simulink model "smart_sensor_Simulation"  (Simulink 6.4)
settings: Solver=FixedStepDiscrete  StartTime=0.0  StopTime=10.0  FixedStep=0.001  RelTol=1e-3
libraries: dsPICdrivers x1, simulink x1
settings Model: Creator=Zion  LastModifiedBy=Lubin
settings OptimizationCC: ExpressionDepthLimit=2147483647  OptimizeModelRefInitCode=on  LifeSpan=1  SimCompilerOptimization=Off
settings DebuggingCC: SignalResolutionControl=UseLocalSettings  MultiTaskDSMMsg=error  MultiTaskCondExecSysMsg=error  StateNameClashWarn=warning
settings HardwareCC: ProdBitPerInt=16  ProdEndianess=LittleEndian  ProdWordSize=16  ProdHWDeviceType=16-bit Generic  TargetHWDeviceType=32-bit Generic
settings RTWCC: SystemTargetFile=dspic.tlc  TemplateMakefile=dspic_pic30_gcc.tmf  PostCodeGenCommand=dsPIC_Compile()  Description=Embedded Target for Microchip dsPIC (real-time)  ProcessScript=dspic_make_rtw_hook  RTWCompilerOptimization=Off
settings CodeAppCC: IgnoreCustomStorageClasses=off
settings STFCustomTargetCC: TargetFcnLib=ansi_tfl_tmw.mat  GenFloatMathFcnCalls=ANSI_C  ModelReferenceCompliant=off  IncludeMdlTerminateFcn=off  CombineOutputUpdateFcns=on  SuppressErrorStatus=on  ERTCustomFileBanners=on  SupportContinuousTime=off  SupportNonInlinedSFcns=off  SystemTargetFile=dspic.tlc
settings ERTTargetCC: TargetFcnLib=ansi_tfl_tmw.mat  GenFloatMathFcnCalls=ANSI_C  ModelReferenceCompliant=off  CompOptLevelCompliant=off  IncludeMdlTerminateFcn=off  SuppressErrorStatus=on  ModelStepFunctionPrototypeControlCompliant=off  InlinedParameterPlacement=NonHierarchical  ERTSrcFileBannerTemplate=dsPIC_code_template.cgt  ERTHdrFileBannerTemplate=dsPIC_code_template.cgt  ERTDataSrcFileTemplate=dsPIC_code_template.cgt  ERTDataHdrFileTemplate=dsPIC_code_template.cgt  ERTCustomFileTemplate=dsPIC_main.tlc
settings CustomProperty: DataType=string  Value=C:\PROGRA~1\MATLAB\R2007b\bin\win32\gmake

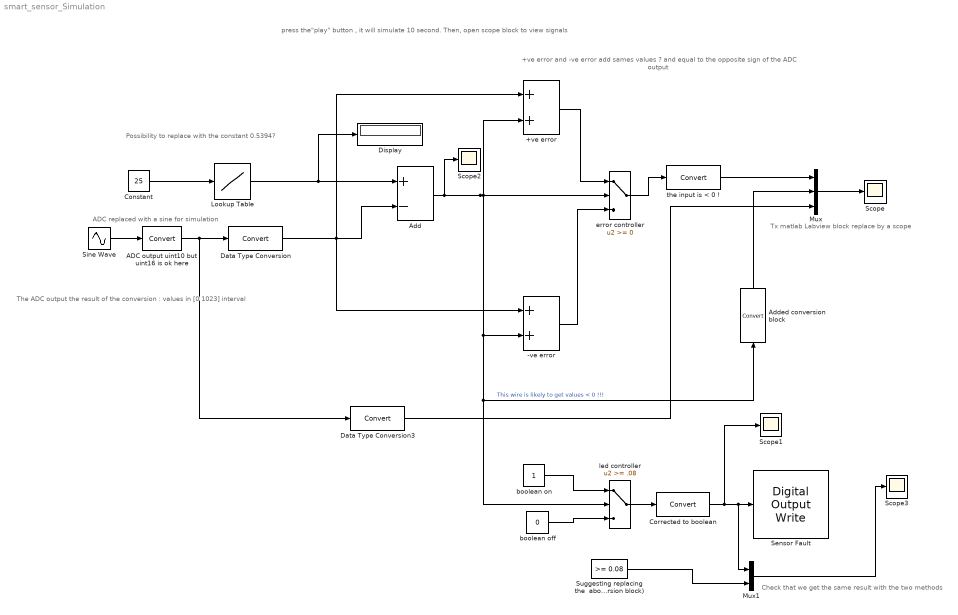
== system smart_sensor_Simulation ==
  note: Possibility to replace with the constant 0.5394?
  note: The ADC output the
      | result of the conversion :
      | values in [0 1023] interval
  note: +ve error and -ve error add sames values ?
      | and equal to the opposite sign of the ADC output
  note: press the"play" button , it will simulate 10 second. Then, open scope block to view signals
  note: ADC replaced with a sine for simulation
  note: Tx matlab Labview block replace by a scope
  note: Check that we get the same result with the two methods
  +ve error : Sum  OutDataTypeMode=double  OutDataType=sfix(16)  OutScaling=2^-10
  -ve error : Sum  OutDataTypeMode=double  OutDataType=sfix(16)  OutScaling=2^-10
  ADC output uint10 but uint16 is ok here : DataTypeConversion  OutDataTypeMode=uint16  OutDataType=sfix(16)  OutScaling=2^0
  Add : Sum  Inputs=+-  OutDataType=sfix(16)  OutScaling=2^-10
  Added conversion block : DataTypeConversion  Orientation=up  OutDataTypeMode=uint16  OutDataType=sfix(16)  OutScaling=2^0
  Constant : Constant  Value=25  OutDataTypeMode=double  OutDataType=sfix(16)  OutScaling=2^0
  Corrected to boolean : DataTypeConversion  OutDataTypeMode=boolean  OutDataType=sfix(16)  OutScaling=2^0
  Data Type Conversion : DataTypeConversion  OutDataTypeMode=double  OutDataType=sfix(16)  OutScaling=2^0
  Data Type Conversion3 : DataTypeConversion  OutDataTypeMode=uint16  OutDataType=sfix(16)  OutScaling=2^0
  Display : Display
  Lookup Table : Lookup  InputValues=[-55 23 150]  OutputValues=[-1.1 .5 3]  LookUpMeth=Interpolation-Use End Values  OutDataTypeMode=double  OutDataType=sfix(16)  OutScaling=2^0
  Mux : Mux  Inputs=3
  Mux1 : Mux  Inputs=2
  Scope{,1..3} (4 alike) : Scope
      Scope2 settings: SaveName=ScopeData2
      Scope3 settings: SaveName=ScopeData3
  Sensor Fault : dsPICdrivers/Digital I//O/Digital Output Write  Tag=dsPIC_Digital_Output  Priority=5  PORT=E  Pin=[0 ]  Simultaneous=off  OrderingInOutPopup=None
  Sine Wave : Sin  Amplitude=511  Bias=512  Frequency=2*pi  SampleTime=.001
  Suggesting replacing the  above blocks with this (replace also the conversion block) : simulink/Logic and Bit Operations/Compare To Constant  SystemSampleTime=-1  relop=>=  const=0.08  LogicOutDataTypeMode=boolean  ZeroCross=off
  boolean off : Constant  Value=0  OutDataTypeMode=double  OutDataType=sfix(16)  OutScaling=2^0
  boolean on : Constant  OutDataTypeMode=double  OutDataType=sfix(16)  OutScaling=2^0
  error controller : Switch  OutDataTypeMode=double
  led controller : Switch  Threshold=.08  OutDataTypeMode=double
  the input is < 0 ! : DataTypeConversion  OutDataTypeMode=uint16  OutDataType=sfix(16)  OutScaling=2^0
  wires:
  Constant/1 -> Lookup Table/1
  Lookup Table/1 -> Add/1, Display/1
  Add/1 -> +ve error/2, -ve error/2, led controller/2, Added conversion block/1, error controller/2, Scope2/1  "This wire is likely to get values < 0 !!!"
  +ve error/1 -> error controller/1
  -ve error/1 -> error controller/3
  Data Type Conversion/1 -> Add/2, +ve error/1, -ve error/1
  Sine Wave/1 -> ADC output uint10 but uint16 is ok here/1
  error controller/1 -> the input is < 0 !/1
  boolean on/1 -> led controller/1
  boolean off/1 -> led controller/3
  led controller/1 -> Corrected to boolean/1
  Corrected to boolean/1 -> Scope1/1, Sensor Fault/1, Mux1/1
  the input is < 0 !/1 -> Mux/1
  Data Type Conversion3/1 -> Mux/3
  Added conversion block/1 -> Mux/2
  Mux/1 -> Scope/1
  ADC output uint10 but uint16 is ok here/1 -> Data Type Conversion/1, Data Type Conversion3/1
  Suggesting replacing the  above blocks with this (replace also the conversion block)/1 -> Mux1/2
  Mux1/1 -> Scope3/1
